simulink model "nmm2d"  (R2025a)
settings: Solver=ode15s  StartTime=0.0  StopTime=20  FixedStep=1e-3  MaxStep=ts_max  RelTol=1e-3  AbsTol=1e-4  EnableMultiTasking=on
values from neighbouring files (symbols this model uses):
  c = 0.05    [nmm2d_mInit.m]
  c_jointstop = 0.3 / (pi/180)    (= 17.1887338539)    [nmm2d_mInit.m]
  D12_F = 0.16    [nmm2d_mInit.m]
  D12_S = L_S    (= 0.5)    [nmm2d_mInit.m]
  D12_T = L_T    (= 0.5)    [nmm2d_mInit.m]
  D1G_F = 0.14    [nmm2d_mInit.m]
  D1G_HAT = 0.35    [nmm2d_mInit.m]
  D1G_S = 0.3    [nmm2d_mInit.m]
  D1G_T = 0.3    [nmm2d_mInit.m]
  DeltaThRef = 5e-3    (= 0.005)    [nmm2d_mInit.m]
  eref = 0.04    [nmm2d_mInit.m]
  FmaxVec = [FmaxSOL FmaxTA FmaxGAS FmaxVAS FmaxHAM FmaxGLU FmaxHFL               FmaxSOL FmaxTA FmaxGAS FmaxVAS FmaxHAM FmaxGLU FmaxHFL]'    [nmm2d_mInit.m]
  g = 9.81    [nmm2d_mInit.m]
  GainDeltaTheta = 2 /100*180/pi    (= 1.14591559026)    [nmm2d_cInit.m]
  GainGAS = 1.1/FmaxGAS    [nmm2d_cInit.m]
  GainGLU = 0.5/FmaxGLU    [nmm2d_cInit.m]
  GainHAM = 0.65/FmaxHAM    [nmm2d_cInit.m]
  GainHAMHFL = 4    [nmm2d_cInit.m]
  GainHFL = 0.5    [nmm2d_cInit.m]
  GainKneOverExt = 2    [nmm2d_cInit.m]
  GainSOL = 1.2/FmaxSOL    [nmm2d_cInit.m]
  GainSOLTA = 0.4/FmaxSOL    [nmm2d_cInit.m]
  GainTA = 1.1    [nmm2d_cInit.m]
  GainVAS = 1.2/FmaxVAS    [nmm2d_cInit.m]
  HAT_CG0 = [-D12_F; 0] + Rot120*[L_S;0] + Rot120*Rot230*[-L_T;0]            + Rot120*Rot230*Rot340*[D1G_HAT;0]    [nmm2d_cInit.m]
  In_F = 0.005    [nmm2d_mInit.m]
  In_HAT = 3    [nmm2d_mInit.m]
  In_S = 0.05    [nmm2d_mInit.m]
  In_T = 0.15    [nmm2d_mInit.m]
  K = 5    [nmm2d_mInit.m]
  k_gx = (2*(m_F+m_S+m_T)+m_HAT)*g/0.1    (= 7848)    [nmm2d_mInit.m]
  k_gy = (2*(m_F+m_S+m_T)+m_HAT)*g/0.01    (= 78480)    [nmm2d_mInit.m]
  k_pressure = m_HAT * 9.81 / DeltaThRef    (= 104967)    [nmm2d_mInit.m]
  K_swing = 0.25    [nmm2d_cInit.m]
  KneePh23Offset = 170*pi/180    (= 2.96705972839)    [nmm2d_cInit.m]
  L_F = 0.2    [nmm2d_mInit.m]
  L_HAT = 0.8    [nmm2d_mInit.m]
  L_S = 0.5    [nmm2d_mInit.m]
  L_T = 0.5    [nmm2d_mInit.m]
  LceOffsetHAM = 0.85    [nmm2d_cInit.m]
  LceOffsetHFL = 0.65    [nmm2d_cInit.m]
  LceOffsetTA = 1-0.5*w    [nmm2d_cInit.m]
  LongDelay = 0.020    (= 0.02)    [nmm2d_cInit.m]
  loptGAS = 0.05    [nmm2d_mInit.m]
  loptGLU = 0.11    [nmm2d_mInit.m]
  loptHAM = 0.10    (= 0.1)    [nmm2d_mInit.m]
  loptHFL = 0.11    [nmm2d_mInit.m]
  loptSOL = 0.04    [nmm2d_mInit.m]
  loptTA = 0.06    [nmm2d_mInit.m]
  loptVAS = 0.08    [nmm2d_mInit.m]
  loptVec = [loptSOL loptTA loptGAS loptVAS loptHAM loptGLU loptHFL               loptSOL loptTA loptGAS loptVAS loptHAM loptGLU loptHFL]'    [nmm2d_mInit.m]
  Lphi120 = 85*pi/180    (= 1.4835298642)    [nmm2d_cInit.m]
  Lphi230 = 175*pi/180    (= 3.05432619099)    [nmm2d_cInit.m]
  Lphi340 = 175*pi/180    (= 3.05432619099)    [nmm2d_cInit.m]
  lslackGAS = 0.40    (= 0.4)    [nmm2d_mInit.m]
  lslackGLU = 0.13    [nmm2d_mInit.m]
  lslackHAM = 0.31    [nmm2d_mInit.m]
  lslackHFL = 0.10    (= 0.1)    [nmm2d_mInit.m]
  lslackSOL = 0.26    [nmm2d_mInit.m]
  lslackTA = 0.24    [nmm2d_mInit.m]
  lslackVAS = 0.23    [nmm2d_mInit.m]
  lslackVec = [lslackSOL lslackTA lslackGAS lslackVAS lslackHAM lslackGLU lslackHFL                 lslackSOL lslackTA lslackGAS lslackVAS lslackHAM lslackGLU lslackHFL]'    [nmm2d_mInit.m]
  m_F = 1.25    [nmm2d_mInit.m]
  m_HAT = 53.5    [nmm2d_mInit.m]
  m_S = 3.5    [nmm2d_mInit.m]
  m_T = 8.5    [nmm2d_mInit.m]
  MidDelay = 0.010    (= 0.01)    [nmm2d_cInit.m]
  mu_slide = 0.8    [nmm2d_mInit.m]
  mu_stick = 0.9    [nmm2d_mInit.m]
  N = 1.5    [nmm2d_mInit.m]
  phi12_LowLimit = 70*pi/180    (= 1.2217304764)    [nmm2d_mInit.m]
  phi12_UpLimit = 130*pi/180    (= 2.26892802759)    [nmm2d_mInit.m]
  phi23_UpLimit = 175*pi/180    (= 3.05432619099)    [nmm2d_mInit.m]
  phi34_UpLimit = 230*pi/180    (= 4.01425727959)    [nmm2d_mInit.m]
  phimaxGASa = 110*pi/180    (= 1.91986217719)    [nmm2d_mInit.m]
  phimaxGASk = 140*pi/180    (= 2.44346095279)    [nmm2d_mInit.m]
  phimaxHAMk = 180*pi/180    (= 3.14159265359)    [nmm2d_mInit.m]
  phimaxSOL = 110*pi/180    (= 1.91986217719)    [nmm2d_mInit.m]
  phimaxTA = 80*pi/180    (= 1.3962634016)    [nmm2d_mInit.m]
  phimaxVAS = 165*pi/180    (= 2.87979326579)    [nmm2d_mInit.m]
  phirefGASa = 80*pi/180    (= 1.3962634016)    [nmm2d_mInit.m]
  phirefGASk = 165*pi/180    (= 2.87979326579)    [nmm2d_mInit.m]
  phirefGLU = 150*pi/180    (= 2.61799387799)    [nmm2d_mInit.m]
  phirefHAMh = 155*pi/180    (= 2.70526034059)    [nmm2d_mInit.m]
  phirefHAMk = 180*pi/180    (= 3.14159265359)    [nmm2d_mInit.m]
  phirefHFL = 180*pi/180    (= 3.14159265359)    [nmm2d_mInit.m]
  phirefSOL = 80*pi/180    (= 1.3962634016)    [nmm2d_mInit.m]
  phirefTA = 110*pi/180    (= 1.91986217719)    [nmm2d_mInit.m]
  phirefVAS = 125*pi/180    (= 2.18166156499)    [nmm2d_mInit.m]
  PosGainGG = 1/(30*pi/180)    (= 1.9098593171)    [nmm2d_cInit.m]
  preA = 0.01    [nmm2d_mInit.m]
  PreStimGAS = 0.01    [nmm2d_cInit.m]
  PreStimGG = 0.05    [nmm2d_cInit.m]
  PreStimGLU = 0.01    [nmm2d_cInit.m]
  PreStimHAM = 0.01    [nmm2d_cInit.m]
  PreStimHFL = 0.01    [nmm2d_cInit.m]
  PreStimSOL = 0.01    [nmm2d_cInit.m]
  PreStimTA = 0.01    [nmm2d_cInit.m]
  PreStimVAS = 0.08    [nmm2d_cInit.m]
  rGASa = 0.05    [nmm2d_mInit.m]
  rGASk = 0.05    [nmm2d_mInit.m]
  rGLU = 0.10    (= 0.1)    [nmm2d_mInit.m]
  rHAMh = 0.08    [nmm2d_mInit.m]
  rHAMk = 0.05    [nmm2d_mInit.m]
  rHFL = 0.10    (= 0.1)    [nmm2d_mInit.m]
  rhoGASa = 0.7    [nmm2d_mInit.m]
  rhoGASk = 0.7    [nmm2d_mInit.m]
  rhoGLU = 0.5    [nmm2d_mInit.m]
  rhoHAMh = 0.7    [nmm2d_mInit.m]
  rhoHAMk = 0.7    [nmm2d_mInit.m]
  rhoHFL = 0.5    [nmm2d_mInit.m]
  rhoSOL = 0.5    [nmm2d_mInit.m]
  rhoTA = 0.7    [nmm2d_mInit.m]
  rhoVAS = 0.7    [nmm2d_mInit.m]
  Rphi120 = 90*pi/180    (= 1.57079632679)    [nmm2d_cInit.m]
  Rphi230 = 175*pi/180    (= 3.05432619099)    [nmm2d_cInit.m]
  Rphi340 = 140*pi/180    (= 2.44346095279)    [nmm2d_cInit.m]
  rSOL = 0.05    [nmm2d_mInit.m]
  rTA = 0.04    [nmm2d_mInit.m]
  rVAS = 0.06    [nmm2d_mInit.m]
  ... (+12 more)
undefined symbols (not defined in the file or in its folder): sgn, X, Y, Z
libraries: sm_lib x70, nesl_utility x67, simulink x27, simulink_extras x6
(part 5 of 5)

== system nmm2d/Body Mechanics Layer/Right Ball Contact/Ground Friction Model ==
  note: Horizontal Ground Friction Model
  note: Vertical Ground Stiction Model
  dy [m] : Inport
  vy [m/s] : Inport  Port=2
  x [m] : Inport  Port=3
  vx [m/s] : Inport  Port=4
  vBelt [m/s] : Inport  Port=5
  Contact! : EnablePort  StatesWhenEnabling=reset
  Data Type Conversion : DataTypeConversion  OutDataTypeStr=double  SaturateOnIntegerOverflow=off  RndMeth=Floor
  Friction Switch : Subsystem
  Gain3 : Gain  Gain=k_gy
  Gain4 : Gain  Gain=1/v_gy_max
  Logical Operator : Logic  Operator=NOT  AllPortsSameDT=off  OutDataTypeStr=boolean
  Mux1 : Mux  Inputs=2
  Sum1 : Sum
  X-Axis Kinetic Friction Model : Subsystem
  X-Axis Static Friction Model : Subsystem
  Y-Axis Ground Force : Fcn  Expr="- u(1)  *  (1-u(2)) * (u(2)<1)"
  Fy_Ground[N] : Outport  OutputWhenDisabled=reset  InitialOutput=0
      settings: AttributesFormatString=initial = '%<InitialOutput>'\nwhen disabled = '%<OutputWhenDisabled>'
  Fx_Friction [N] : Outport  Port=2  OutputWhenDisabled=reset  InitialOutput=0
      settings: AttributesFormatString=initial = '%<InitialOutput>'\nwhen\ndisabled\n'%<OutputWhenDisabled>'
  Stiction! : Outport  Port=3  OutputWhenDisabled=reset  InitialOutput=0
      settings: AttributesFormatString=initial = '%<InitialOutput>'\nwhen\ndisabled\n'%<OutputWhenDisabled>'
  wires:
  Y-Axis Ground Force/1 -> X-Axis Kinetic Friction Model/4(F_Normal [N]), X-Axis Static Friction Model/1(F_Normal [N]), Fy_Ground[N]/1
  dy [m]/1 -> Gain3/1
  vy [m/s]/1 -> Gain4/1
  x [m]/1 -> X-Axis Kinetic Friction Model/1(pos [m]), X-Axis Static Friction Model/3(pos [m])
  vx [m/s]/1 -> X-Axis Static Friction Model/4(vel [m/s]), X-Axis Kinetic Friction Model/2(vel [m/s])
  X-Axis Kinetic Friction Model/1(initial posFP [m]) -> X-Axis Static Friction Model/5(initial posFP [m])
  X-Axis Kinetic Friction Model/3(F_Slide [N]) -> Sum1/2
  X-Axis Static Friction Model/1(F_Stick [N]) -> Sum1/1
  Sum1/1 -> Fx_Friction [N]/1
  Friction Switch/1(Stiction) -> X-Axis Static Friction Model/Enable, Logical Operator/1, Data Type Conversion/1
  X-Axis Static Friction Model/2(Sliding!) -> Friction Switch/1(Slide!)
  X-Axis Kinetic Friction Model/2(Stiction!) -> Friction Switch/2(Stick!)
  Logical Operator/1 -> X-Axis Kinetic Friction Model/Enable
  Data Type Conversion/1 -> Stiction!/1
  Mux1/1 -> Y-Axis Ground Force/1
  Gain3/1 -> Mux1/1
  Gain4/1 -> Mux1/2
  vBelt [m/s]/1 -> X-Axis Kinetic Friction Model/3(vBelt [m/s]), X-Axis Static Friction Model/2(vBelt [m/s])

== system nmm2d/Body Mechanics Layer/Right Heel Contact/Ground Friction Model ==
  note: Vertical Ground Stiction Model
  note: Horizontal Ground Friction Model
  dy [m] : Inport
  vy [m/s] : Inport  Port=2
  x [m] : Inport  Port=3
  vx [m/s] : Inport  Port=4
  vBelt [m/s] : Inport  Port=5
  Contact! : EnablePort  StatesWhenEnabling=reset
  Data Type Conversion : DataTypeConversion  OutDataTypeStr=double  SaturateOnIntegerOverflow=off  RndMeth=Floor
  Friction Switch : Subsystem
  Gain3 : Gain  Gain=k_gy
  Gain4 : Gain  Gain=1/v_gy_max
  Logical Operator : Logic  Operator=NOT  AllPortsSameDT=off  OutDataTypeStr=boolean
  Mux1 : Mux  Inputs=2
  Sum1 : Sum
  X-Axis Kinetic Friction Model : Subsystem
  X-Axis Static Friction Model : Subsystem
  Y-Axis Ground Force : Fcn  Expr="- u(1)  *  (1-u(2)) * (u(2)<1)"
  Fy_Ground[N] : Outport  OutputWhenDisabled=reset  InitialOutput=0
      settings: AttributesFormatString=initial = '%<InitialOutput>'\nwhen disabled = '%<OutputWhenDisabled>'
  Fx_Friction [N] : Outport  Port=2  OutputWhenDisabled=reset  InitialOutput=0
      settings: AttributesFormatString=initial = '%<InitialOutput>'\nwhen\ndisabled\n'%<OutputWhenDisabled>'
  Stiction! : Outport  Port=3  OutputWhenDisabled=reset  InitialOutput=0
      settings: AttributesFormatString=initial = '%<InitialOutput>'\nwhen\ndisabled\n'%<OutputWhenDisabled>'
  wires:
  vBelt [m/s]/1 -> X-Axis Static Friction Model/2(vBelt [m/s]), X-Axis Kinetic Friction Model/3(vBelt [m/s])
  Gain4/1 -> Mux1/2
  Gain3/1 -> Mux1/1
  Mux1/1 -> Y-Axis Ground Force/1
  Data Type Conversion/1 -> Stiction!/1
  Logical Operator/1 -> X-Axis Kinetic Friction Model/Enable
  X-Axis Kinetic Friction Model/2(Stiction!) -> Friction Switch/2(Stick!)
  X-Axis Static Friction Model/2(Sliding!) -> Friction Switch/1(Slide!)
  Friction Switch/1(Stiction) -> Data Type Conversion/1, Logical Operator/1, X-Axis Static Friction Model/Enable
  Sum1/1 -> Fx_Friction [N]/1
  X-Axis Static Friction Model/1(F_Stick [N]) -> Sum1/1
  X-Axis Kinetic Friction Model/3(F_Slide [N]) -> Sum1/2
  X-Axis Kinetic Friction Model/1(initial posFP [m]) -> X-Axis Static Friction Model/5(initial posFP [m])
  vx [m/s]/1 -> X-Axis Kinetic Friction Model/2(vel [m/s]), X-Axis Static Friction Model/4(vel [m/s])
  x [m]/1 -> X-Axis Static Friction Model/3(pos [m]), X-Axis Kinetic Friction Model/1(pos [m])
  vy [m/s]/1 -> Gain4/1
  dy [m]/1 -> Gain3/1
  Y-Axis Ground Force/1 -> Fy_Ground[N]/1, X-Axis Static Friction Model/1(F_Normal [N]), X-Axis Kinetic Friction Model/4(F_Normal [N])

== system nmm2d/Muscle Actuation Layer/VECTORIZED Muscle Dynamics/BE force-length relation ==
  note: Buffer Elasticity BE
  lce [lopt] : Inport
  Constant1 : Constant  Value=1-w
  Math Function : Math  Operator=square  SignedPower=on
  Sum4 : Sum  Inputs=|+-  InputSameDT=on  SaturateOnIntegerOverflow=on  OutDataTypeStr=Inherit: Same as first input
  buffer engaged? : simulink/Logic and Bit Operations/Compare To Zero  relop=<  OutDataTypeStr=boolean  ZeroCross=off
  force of buffer elasticity : Product  Inputs=**
  reference strain [lslack] : Constant  Value=w/2
  relative strain : Product  Inputs=*/
  fbe [Fmax] : Outport
  wires:
  force of buffer elasticity/1 -> fbe [Fmax]/1
  Math Function/1 -> force of buffer elasticity/2
  buffer engaged?/1 -> force of buffer elasticity/1
  Constant1/1 -> Sum4/2
  Sum4/1 -> relative strain/1, buffer engaged?/1
  reference strain [lslack]/1 -> relative strain/2
  relative strain/1 -> Math Function/1
  lce [lopt]/1 -> Sum4/1

== system nmm2d/Muscle Actuation Layer/VECTORIZED Muscle Dynamics/CE force-length relation ==
  note: CE Force-Length Relationship
  lce [lopt] : Inport
  Abs : Abs  SaturateOnIntegerOverflow=off
  Constant1 : Constant
  Constant2 : Constant  Value=3
  Gain : Gain  Gain=log(c)
  Math Function : Math  SignedPower=on
  Math Function1 : Math  Operator=pow  SignedPower=on
  Sum4 : Sum  Inputs=|+-  InputSameDT=on  SaturateOnIntegerOverflow=on  OutDataTypeStr=Inherit: Same as first input
  normalized position : Product  Inputs=*/
  relative width : Constant  Value=w
  fce [Fmax] : Outport
  wires:
  Math Function/1 -> fce [Fmax]/1
  Gain/1 -> Math Function/1
  Math Function1/1 -> Gain/1
  Constant2/1 -> Math Function1/2
  normalized position/1 -> Math Function1/1
  Abs/1 -> normalized position/1
  Sum4/1 -> Abs/1
  Constant1/1 -> Sum4/2
  relative width/1 -> normalized position/2
  lce [lopt]/1 -> Sum4/1

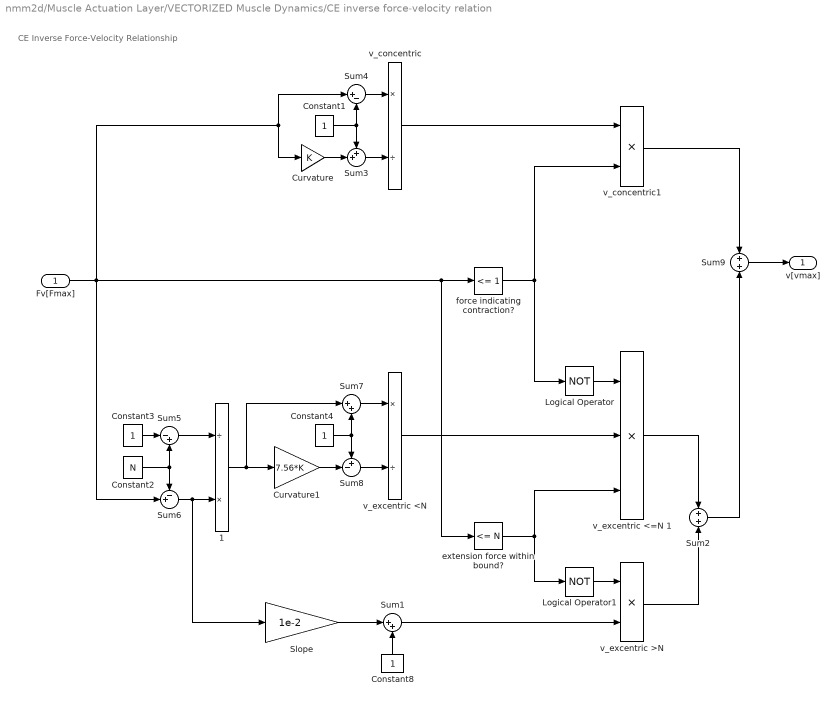
== system nmm2d/Muscle Actuation Layer/VECTORIZED Muscle Dynamics/CE inverse force-velocity relation ==
  note: CE Inverse Force-Velocity Relationship
  Fv[Fmax] : Inport
  1 : Product  Inputs=/*
  Constant{1,3..4,8} (4 alike) : Constant
  Constant2 : Constant  Value=N
  Curvature : Gain  Gain=K  SaturateOnIntegerOverflow=on  OutDataTypeStr=Inherit: Same as input  ParamDataTypeStr=Inherit: Same as input
  Curvature1 : Gain  Gain=7.56*K  SaturateOnIntegerOverflow=on  OutDataTypeStr=Inherit: Same as input  ParamDataTypeStr=Inherit: Same as input
  Logical Operator : Logic  Operator=NOT  AllPortsSameDT=off  OutDataTypeStr=boolean
  Logical Operator1 : Logic  Operator=NOT  AllPortsSameDT=off  OutDataTypeStr=boolean
  Slope : Gain  Gain=1e-2  SaturateOnIntegerOverflow=on  OutDataTypeStr=Inherit: Same as input  ParamDataTypeStr=Inherit: Same as input
  Sum1 : Sum  Inputs=|++  InputSameDT=on  SaturateOnIntegerOverflow=on  OutDataTypeStr=Inherit: Same as first input
  Sum2 : Sum  InputSameDT=on  SaturateOnIntegerOverflow=on  OutDataTypeStr=Inherit: Same as first input
  Sum3 : Sum  Inputs=++|  InputSameDT=on  SaturateOnIntegerOverflow=on  OutDataTypeStr=Inherit: Same as first input
  Sum4 : Sum  Inputs=|+-  InputSameDT=on  SaturateOnIntegerOverflow=on  OutDataTypeStr=Inherit: Same as first input
  Sum5 : Sum  Inputs=|-+  InputSameDT=on  SaturateOnIntegerOverflow=on  OutDataTypeStr=Inherit: Same as first input
  Sum6 : Sum  Inputs=-+|  InputSameDT=on  SaturateOnIntegerOverflow=on  OutDataTypeStr=Inherit: Same as first input
  Sum7 : Sum  Inputs=|++  InputSameDT=on  SaturateOnIntegerOverflow=on  OutDataTypeStr=Inherit: Same as first input
  Sum8 : Sum  Inputs=+-|  InputSameDT=on  SaturateOnIntegerOverflow=on  OutDataTypeStr=Inherit: Same as first input
  Sum9 : Sum  InputSameDT=on  SaturateOnIntegerOverflow=on  OutDataTypeStr=Inherit: Same as first input
  extension force within bound? : simulink/Logic and Bit Operations/Compare To Constant  relop=<=  const=N  OutDataTypeStr=boolean  ZeroCross=off
  force indicating contraction? : simulink/Logic and Bit Operations/Compare To Constant  relop=<=  const=1  OutDataTypeStr=boolean  ZeroCross=off
  v_concentric : Product  Inputs=*/
  v_concentric1 : Product  Inputs=**
  v_excentric <=N 1 : Product  Inputs=***
  v_excentric <N : Product  Inputs=*/
  v_excentric >N : Product  Inputs=**
  v[vmax] : Outport
  wires:
  Sum2/1 -> Sum9/2
  v_excentric <=N 1/1 -> Sum2/1
  Logical Operator1/1 -> v_excentric >N/1
  v_excentric >N/1 -> Sum2/2
  Logical Operator/1 -> v_excentric <=N 1/1
  Fv[Fmax]/1 -> Sum6/2, extension force within bound?/1, force indicating contraction?/1, Curvature/1, Sum4/1
  extension force within bound?/1 -> Logical Operator1/1, v_excentric <=N 1/3
  force indicating contraction?/1 -> Logical Operator/1, v_concentric1/2
  Sum1/1 -> v_excentric >N/2
  v_concentric1/1 -> Sum9/1
  v_excentric <N/1 -> v_excentric <=N 1/2
  Constant3/1 -> Sum5/1
  Sum5/1 -> 1/1
  Constant2/1 -> Sum5/2, Sum6/1
  Sum6/1 -> Slope/1, 1/2
  Constant8/1 -> Sum1/2
  Slope/1 -> Sum1/1
  Sum9/1 -> v[vmax]/1
  v_concentric/1 -> v_concentric1/1
  Sum7/1 -> v_excentric <N/1
  Sum8/1 -> v_excentric <N/2
  Curvature1/1 -> Sum8/2
  Constant4/1 -> Sum8/1, Sum7/2
  1/1 -> Curvature1/1, Sum7/1
  Sum3/1 -> v_concentric/2
  Sum4/1 -> v_concentric/1
  Constant1/1 -> Sum3/1, Sum4/2
  Curvature/1 -> Sum3/2

== system nmm2d/Muscle Actuation Layer/VECTORIZED Muscle Dynamics/PE force-length relation ==
  note: Parallel Elasticity PE
  lce [lopt] : Inport
  Constant3 : Constant
  Math Function2 : Math  Operator=square  SignedPower=on
  Sum1 : Sum  Inputs=|+-  InputSameDT=on  SaturateOnIntegerOverflow=on  OutDataTypeStr=Inherit: Same as first input
  force of buffer elasticity : Product  Inputs=**
  parallel elasticity engaged? : simulink/Logic and Bit Operations/Compare To Zero  relop=>  OutDataTypeStr=boolean  ZeroCross=off
  reference strain [lopt] : Constant  Value=w
  relative strain : Product  Inputs=*/
  fpe [Fmax] : Outport
  wires:
  parallel elasticity engaged?/1 -> force of buffer elasticity/1
  force of buffer elasticity/1 -> fpe [Fmax]/1
  Math Function2/1 -> force of buffer elasticity/2
  relative strain/1 -> Math Function2/1
  reference strain [lopt]/1 -> relative strain/2
  Sum1/1 -> relative strain/1, parallel elasticity engaged?/1
  Constant3/1 -> Sum1/2
  lce [lopt]/1 -> Sum1/1

== system nmm2d/Muscle Actuation Layer/VECTORIZED Muscle Dynamics/SE force-length relation ==
  note: SE Force-Length Relationship
  lse [lslack] : Inport
  Constant1 : Constant
  Math Function : Math  Operator=square  SignedPower=on
  Sum4 : Sum  Inputs=|+-  InputSameDT=on  SaturateOnIntegerOverflow=on  OutDataTypeStr=Inherit: Same as first input
  force above slack length : Product  Inputs=**
  greater than slack length? : simulink/Logic and Bit Operations/Compare To Zero  relop=>  OutDataTypeStr=boolean  ZeroCross=off
  reference strain [lslack] : Constant  Value=eref
  relative strain : Product  Inputs=*/
  fse [Fmax] : Outport
  wires:
  force above slack length/1 -> fse [Fmax]/1
  greater than slack length?/1 -> force above slack length/1
  Constant1/1 -> Sum4/2
  Sum4/1 -> relative strain/1, greater than slack length?/1
  reference strain [lslack]/1 -> relative strain/2
  relative strain/1 -> Math Function/1
  lse [lslack]/1 -> Sum4/1
  Math Function/1 -> force above slack length/2

== system nmm2d/Body Mechanics Layer/Left Ball Contact/Ground Friction Model/Friction Switch ==
  note: Static/Kinetic Friction Switch
  Slide! : Inport
  Stick! : Inport  Port=2
  Memory : Memory
  S-R Flip-Flop : simulink_extras/Flip Flops/S-R Flip-Flop  initial_condition=1
  Terminator : Terminator
  Stiction : Outport
  wires:
  S-R Flip-Flop/1 -> Memory/1
  S-R Flip-Flop/2 -> Terminator/1
  Stick!/1 -> S-R Flip-Flop/1
  Slide!/1 -> S-R Flip-Flop/2
  Memory/1 -> Stiction/1

== system nmm2d/Body Mechanics Layer/Left Ball Contact/Ground Friction Model/X-Axis Kinetic Friction Model ==
  note: Kinetic Friction Model
  note: Footpoint Determiner
  note: Sliding Limit Detector
  pos [m] : Inport
  vel [m/s] : Inport  Port=2
  vBelt [m/s] : Inport  Port=3
  F_Normal [N] : Inport  Port=4
  Enable : EnablePort  StatesWhenEnabling=reset  ZeroCross=off
  Abs : Abs  SaturateOnIntegerOverflow=off
  Constant : Constant  Value=vLimit
  FixPt Relational Operator : RelationalOperator  Operator=>  OutDataTypeStr=boolean  ZeroCross=off  InputSameDT=off
  Memory : Memory
  Negative : simulink/Logic and Bit Operations/Compare To Zero  relop=<  OutDataTypeStr=boolean
  Product : Product  RndMeth=Zero
  Sign1 : Signum
  Sum : Sum  Inputs=|+-
  Sum1 : Sum  Inputs=|+-
  reverse : Gain  Gain=-1
  sliding friction coefficient : Gain  Gain=mu_slide
  initial posFP [m] : Outport  InitialOutput=0
      settings: AttributesFormatString=initial = '%<InitialOutput>'\nwhen disabled = '%<OutputWhenDisabled>'
  Stiction! : Outport  Port=2  OutputWhenDisabled=reset  InitialOutput=0
      settings: AttributesFormatString=initial = '%<InitialOutput>'\nwhen disabled = '%<OutputWhenDisabled>'
  F_Slide [N] : Outport  Port=3  OutputWhenDisabled=reset  InitialOutput=0
      settings: AttributesFormatString=initial = '%<InitialOutput>'\nwhen disabled = '%<OutputWhenDisabled>'
  wires:
  reverse/1 -> Product/1
  F_Normal [N]/1 -> sliding friction coefficient/1
  Sum1/1 -> Sign1/1, Abs/1
  pos [m]/1 -> initial posFP [m]/1
  Product/1 -> F_Slide [N]/1
  sliding friction coefficient/1 -> Product/2
  Sign1/1 -> reverse/1
  FixPt Relational Operator/1 -> Stiction!/1
  Memory/1 -> FixPt Relational Operator/2
  Negative/1 -> FixPt Relational Operator/1, Memory/1
  Abs/1 -> Sum/1
  Sum/1 -> Negative/1
  Constant/1 -> Sum/2
  vel [m/s]/1 -> Sum1/1
  vBelt [m/s]/1 -> Sum1/2

== system nmm2d/Body Mechanics Layer/Left Ball Contact/Ground Friction Model/X-Axis Static Friction Model ==
  note: Zero multiplication prevents
      | horizontal friction model from
      | oscillating between static and kinetic
      | friction when the vertical force is zero but
      | the ground level is not yet reached
      | in the upward motion
  note: Stiction Limit Detector
  note: Static Friction Model
  F_Normal [N] : Inport
  vBelt [m/s] : Inport  Port=2
  pos [m] : Inport  Port=3
  vel [m/s] : Inport  Port=4
  initial posFP [m] : Inport  Port=5
  Enable : EnablePort  StatesWhenEnabling=reset  ZeroCross=off
  Abs : Abs  SaturateOnIntegerOverflow=off
  Abs. : Abs  SaturateOnIntegerOverflow=off
  Check Vertical Friction : Product  RndMeth=Zero
  FixPt Relational Operator : RelationalOperator  Operator=>  OutDataTypeStr=boolean  ZeroCross=off  InputSameDT=off
  Gain3 : Gain  Gain=k_gx
  Gain4 : Gain  Gain=1/v_gx_max
  Integrator : Integrator  InitialConditionSource=external
  Memory : Memory
  Mux1 : Mux  Inputs=2
  Positive : simulink/Logic and Bit Operations/Compare To Zero  relop=>  OutDataTypeStr=boolean
  Positive1 : simulink/Logic and Bit Operations/Compare To Zero  relop=>  OutDataTypeStr=boolean
  Sum : Sum  Inputs=-+
  Sum1 : Sum  Inputs=-+|
  Sum2 : Sum  Inputs=-+|
  X-Axis Stiction Force : Fcn  Expr=-u(1) * (1+sgn(u(1))*u(2))
  stiction limit force : Gain  Gain=mu_stick
  F_Stick [N] : Outport  OutputWhenDisabled=reset  InitialOutput=0
      settings: AttributesFormatString=when disabled: %<OutputWhenDisabled>\ninitial: %<InitialOutput>
  Sliding! : Outport  Port=2  OutputWhenDisabled=reset  InitialOutput=0
      settings: AttributesFormatString=when disabled: %<OutputWhenDisabled>\ninitial: %<InitialOutput>
  wires:
  Check Vertical Friction/1 -> Abs./1, F_Stick [N]/1
  Positive1/1 -> Check Vertical Friction/2
  X-Axis Stiction Force/1 -> Check Vertical Friction/1
  stiction limit force/1 -> Abs/1
  Abs/1 -> Sum/1
  FixPt Relational Operator/1 -> Sliding!/1
  Gain4/1 -> Mux1/2
  Gain3/1 -> Mux1/1
  Mux1/1 -> X-Axis Stiction Force/1
  Abs./1 -> Sum/2
  Positive/1 -> Memory/1, FixPt Relational Operator/1
  Memory/1 -> FixPt Relational Operator/2
  Sum/1 -> Positive/1
  pos [m]/1 -> Sum2/2
  Sum2/1 -> Gain3/1  "dx"
  F_Normal [N]/1 -> Positive1/1, stiction limit force/1
  initial posFP [m]/1 -> Integrator/2
  vBelt [m/s]/1 -> Sum1/1, Integrator/1
  Integrator/1 -> Sum2/1  "xFP"
  vel [m/s]/1 -> Sum1/2
  Sum1/1 -> Gain4/1  "dx"

== system nmm2d/Body Mechanics Layer/Left Heel Contact/Ground Friction Model/Friction Switch ==
  note: Static/Kinetic Friction Switch
  Slide! : Inport
  Stick! : Inport  Port=2
  Memory : Memory
  S-R Flip-Flop : simulink_extras/Flip Flops/S-R Flip-Flop  initial_condition=1
  Terminator : Terminator
  Stiction : Outport
  wires:
  Memory/1 -> Stiction/1
  Slide!/1 -> S-R Flip-Flop/2
  Stick!/1 -> S-R Flip-Flop/1
  S-R Flip-Flop/2 -> Terminator/1
  S-R Flip-Flop/1 -> Memory/1

== system nmm2d/Body Mechanics Layer/Left Heel Contact/Ground Friction Model/X-Axis Kinetic Friction Model ==
  note: Sliding Limit Detector
  note: Footpoint Determiner
  note: Kinetic Friction Model
  pos [m] : Inport
  vel [m/s] : Inport  Port=2
  vBelt [m/s] : Inport  Port=3
  F_Normal [N] : Inport  Port=4
  Enable : EnablePort  StatesWhenEnabling=reset  ZeroCross=off
  Abs : Abs  SaturateOnIntegerOverflow=off
  Constant : Constant  Value=vLimit
  FixPt Relational Operator : RelationalOperator  Operator=>  OutDataTypeStr=boolean  ZeroCross=off  InputSameDT=off
  Memory : Memory
  Negative : simulink/Logic and Bit Operations/Compare To Zero  relop=<  OutDataTypeStr=boolean
  Product : Product  RndMeth=Zero
  Sign1 : Signum
  Sum : Sum  Inputs=|+-
  Sum1 : Sum  Inputs=|+-
  reverse : Gain  Gain=-1
  sliding friction coefficient : Gain  Gain=mu_slide
  initial posFP [m] : Outport  InitialOutput=0
      settings: AttributesFormatString=initial = '%<InitialOutput>'\nwhen disabled = '%<OutputWhenDisabled>'
  Stiction! : Outport  Port=2  OutputWhenDisabled=reset  InitialOutput=0
      settings: AttributesFormatString=initial = '%<InitialOutput>'\nwhen disabled = '%<OutputWhenDisabled>'
  F_Slide [N] : Outport  Port=3  OutputWhenDisabled=reset  InitialOutput=0
      settings: AttributesFormatString=initial = '%<InitialOutput>'\nwhen disabled = '%<OutputWhenDisabled>'
  wires:
  vBelt [m/s]/1 -> Sum1/2
  vel [m/s]/1 -> Sum1/1
  Constant/1 -> Sum/2
  Sum/1 -> Negative/1
  Abs/1 -> Sum/1
  Negative/1 -> Memory/1, FixPt Relational Operator/1
  Memory/1 -> FixPt Relational Operator/2
  FixPt Relational Operator/1 -> Stiction!/1
  Sign1/1 -> reverse/1
  sliding friction coefficient/1 -> Product/2
  Product/1 -> F_Slide [N]/1
  pos [m]/1 -> initial posFP [m]/1
  Sum1/1 -> Abs/1, Sign1/1
  F_Normal [N]/1 -> sliding friction coefficient/1
  reverse/1 -> Product/1

== system nmm2d/Body Mechanics Layer/Left Heel Contact/Ground Friction Model/X-Axis Static Friction Model ==
  note: Static Friction Model
  note: Stiction Limit Detector
  note: Zero multiplication prevents
      | horizontal friction model from
      | oscillating between static and kinetic
      | friction when the vertical force is zero but
      | the ground level is not yet reached
      | in the upward motion
  F_Normal [N] : Inport
  vBelt [m/s] : Inport  Port=2
  pos [m] : Inport  Port=3
  vel [m/s] : Inport  Port=4
  initial posFP [m] : Inport  Port=5
  Enable : EnablePort  StatesWhenEnabling=reset  ZeroCross=off
  Abs : Abs  SaturateOnIntegerOverflow=off
  Abs. : Abs  SaturateOnIntegerOverflow=off
  Check Vertical Friction : Product  RndMeth=Zero
  FixPt Relational Operator : RelationalOperator  Operator=>  OutDataTypeStr=boolean  ZeroCross=off  InputSameDT=off
  Gain3 : Gain  Gain=k_gx
  Gain4 : Gain  Gain=1/v_gx_max
  Integrator : Integrator  InitialConditionSource=external
  Memory : Memory
  Mux1 : Mux  Inputs=2
  Positive : simulink/Logic and Bit Operations/Compare To Zero  relop=>  OutDataTypeStr=boolean
  Positive1 : simulink/Logic and Bit Operations/Compare To Zero  relop=>  OutDataTypeStr=boolean
  Sum : Sum  Inputs=-+
  Sum1 : Sum  Inputs=-+|
  Sum2 : Sum  Inputs=-+|
  X-Axis Stiction Force : Fcn  Expr=-u(1) * (1+sgn(u(1))*u(2))
  stiction limit force : Gain  Gain=mu_stick
  F_Stick [N] : Outport  OutputWhenDisabled=reset  InitialOutput=0
      settings: AttributesFormatString=when disabled: %<OutputWhenDisabled>\ninitial: %<InitialOutput>
  Sliding! : Outport  Port=2  OutputWhenDisabled=reset  InitialOutput=0
      settings: AttributesFormatString=when disabled: %<OutputWhenDisabled>\ninitial: %<InitialOutput>
  wires:
  Sum1/1 -> Gain4/1  "dx"
  vel [m/s]/1 -> Sum1/2
  Integrator/1 -> Sum2/1  "xFP"
  vBelt [m/s]/1 -> Integrator/1, Sum1/1
  initial posFP [m]/1 -> Integrator/2
  F_Normal [N]/1 -> stiction limit force/1, Positive1/1
  Sum2/1 -> Gain3/1  "dx"
  pos [m]/1 -> Sum2/2
  Sum/1 -> Positive/1
  Memory/1 -> FixPt Relational Operator/2
  Positive/1 -> FixPt Relational Operator/1, Memory/1
  Abs./1 -> Sum/2
  Mux1/1 -> X-Axis Stiction Force/1
  Gain3/1 -> Mux1/1
  Gain4/1 -> Mux1/2
  FixPt Relational Operator/1 -> Sliding!/1
  Abs/1 -> Sum/1
  stiction limit force/1 -> Abs/1
  X-Axis Stiction Force/1 -> Check Vertical Friction/1
  Positive1/1 -> Check Vertical Friction/2
  Check Vertical Friction/1 -> F_Stick [N]/1, Abs./1

== system nmm2d/Body Mechanics Layer/Right Ball Contact/Ground Friction Model/Friction Switch ==
  note: Static/Kinetic Friction Switch
  Slide! : Inport
  Stick! : Inport  Port=2
  Memory : Memory
  S-R Flip-Flop : simulink_extras/Flip Flops/S-R Flip-Flop  initial_condition=1
  Terminator : Terminator
  Stiction : Outport
  wires:
  S-R Flip-Flop/1 -> Memory/1
  S-R Flip-Flop/2 -> Terminator/1
  Stick!/1 -> S-R Flip-Flop/1
  Slide!/1 -> S-R Flip-Flop/2
  Memory/1 -> Stiction/1

== system nmm2d/Body Mechanics Layer/Right Ball Contact/Ground Friction Model/X-Axis Kinetic Friction Model ==
  note: Kinetic Friction Model
  note: Footpoint Determiner
  note: Sliding Limit Detector
  pos [m] : Inport
  vel [m/s] : Inport  Port=2
  vBelt [m/s] : Inport  Port=3
  F_Normal [N] : Inport  Port=4
  Enable : EnablePort  StatesWhenEnabling=reset  ZeroCross=off
  Abs : Abs  SaturateOnIntegerOverflow=off
  Constant : Constant  Value=vLimit
  FixPt Relational Operator : RelationalOperator  Operator=>  OutDataTypeStr=boolean  ZeroCross=off  InputSameDT=off
  Memory : Memory
  Negative : simulink/Logic and Bit Operations/Compare To Zero  relop=<  OutDataTypeStr=boolean
  Product : Product  RndMeth=Zero
  Sign1 : Signum
  Sum : Sum  Inputs=|+-
  Sum1 : Sum  Inputs=|+-
  reverse : Gain  Gain=-1
  sliding friction coefficient : Gain  Gain=mu_slide
  initial posFP [m] : Outport  InitialOutput=0
      settings: AttributesFormatString=initial = '%<InitialOutput>'\nwhen disabled = '%<OutputWhenDisabled>'
  Stiction! : Outport  Port=2  OutputWhenDisabled=reset  InitialOutput=0
      settings: AttributesFormatString=initial = '%<InitialOutput>'\nwhen disabled = '%<OutputWhenDisabled>'
  F_Slide [N] : Outport  Port=3  OutputWhenDisabled=reset  InitialOutput=0
      settings: AttributesFormatString=initial = '%<InitialOutput>'\nwhen disabled = '%<OutputWhenDisabled>'
  wires:
  reverse/1 -> Product/1
  F_Normal [N]/1 -> sliding friction coefficient/1
  Sum1/1 -> Sign1/1, Abs/1
  pos [m]/1 -> initial posFP [m]/1
  Product/1 -> F_Slide [N]/1
  sliding friction coefficient/1 -> Product/2
  Sign1/1 -> reverse/1
  FixPt Relational Operator/1 -> Stiction!/1
  Memory/1 -> FixPt Relational Operator/2
  Negative/1 -> FixPt Relational Operator/1, Memory/1
  Abs/1 -> Sum/1
  Sum/1 -> Negative/1
  Constant/1 -> Sum/2
  vel [m/s]/1 -> Sum1/1
  vBelt [m/s]/1 -> Sum1/2

== system nmm2d/Body Mechanics Layer/Right Ball Contact/Ground Friction Model/X-Axis Static Friction Model ==
  note: Zero multiplication prevents
      | horizontal friction model from
      | oscillating between static and kinetic
      | friction when the vertical force is zero but
      | the ground level is not yet reached
      | in the upward motion
  note: Stiction Limit Detector
  note: Static Friction Model
  F_Normal [N] : Inport
  vBelt [m/s] : Inport  Port=2
  pos [m] : Inport  Port=3
  vel [m/s] : Inport  Port=4
  initial posFP [m] : Inport  Port=5
  Enable : EnablePort  StatesWhenEnabling=reset  ZeroCross=off
  Abs : Abs  SaturateOnIntegerOverflow=off
  Abs. : Abs  SaturateOnIntegerOverflow=off
  Check Vertical Friction : Product  RndMeth=Zero
  FixPt Relational Operator : RelationalOperator  Operator=>  OutDataTypeStr=boolean  ZeroCross=off  InputSameDT=off
  Gain3 : Gain  Gain=k_gx
  Gain4 : Gain  Gain=1/v_gx_max
  Integrator : Integrator  InitialConditionSource=external
  Memory : Memory
  Mux1 : Mux  Inputs=2
  Positive : simulink/Logic and Bit Operations/Compare To Zero  relop=>  OutDataTypeStr=boolean
  Positive1 : simulink/Logic and Bit Operations/Compare To Zero  relop=>  OutDataTypeStr=boolean
  Sum : Sum  Inputs=-+
  Sum1 : Sum  Inputs=-+|
  Sum2 : Sum  Inputs=-+|
  X-Axis Stiction Force : Fcn  Expr=-u(1) * (1+sgn(u(1))*u(2))
  stiction limit force : Gain  Gain=mu_stick
  F_Stick [N] : Outport  OutputWhenDisabled=reset  InitialOutput=0
      settings: AttributesFormatString=when disabled: %<OutputWhenDisabled>\ninitial: %<InitialOutput>
  Sliding! : Outport  Port=2  OutputWhenDisabled=reset  InitialOutput=0
      settings: AttributesFormatString=when disabled: %<OutputWhenDisabled>\ninitial: %<InitialOutput>
  wires:
  Check Vertical Friction/1 -> Abs./1, F_Stick [N]/1
  Positive1/1 -> Check Vertical Friction/2
  X-Axis Stiction Force/1 -> Check Vertical Friction/1
  stiction limit force/1 -> Abs/1
  Abs/1 -> Sum/1
  FixPt Relational Operator/1 -> Sliding!/1
  Gain4/1 -> Mux1/2
  Gain3/1 -> Mux1/1
  Mux1/1 -> X-Axis Stiction Force/1
  Abs./1 -> Sum/2
  Positive/1 -> Memory/1, FixPt Relational Operator/1
  Memory/1 -> FixPt Relational Operator/2
  Sum/1 -> Positive/1
  pos [m]/1 -> Sum2/2
  Sum2/1 -> Gain3/1  "dx"
  F_Normal [N]/1 -> Positive1/1, stiction limit force/1
  initial posFP [m]/1 -> Integrator/2
  vBelt [m/s]/1 -> Sum1/1, Integrator/1
  Integrator/1 -> Sum2/1  "xFP"
  vel [m/s]/1 -> Sum1/2
  Sum1/1 -> Gain4/1  "dx"

== system nmm2d/Body Mechanics Layer/Right Heel Contact/Ground Friction Model/Friction Switch ==
  note: Static/Kinetic Friction Switch
  Slide! : Inport
  Stick! : Inport  Port=2
  Memory : Memory
  S-R Flip-Flop : simulink_extras/Flip Flops/S-R Flip-Flop  initial_condition=1
  Terminator : Terminator
  Stiction : Outport
  wires:
  Memory/1 -> Stiction/1
  Slide!/1 -> S-R Flip-Flop/2
  Stick!/1 -> S-R Flip-Flop/1
  S-R Flip-Flop/2 -> Terminator/1
  S-R Flip-Flop/1 -> Memory/1

== system nmm2d/Body Mechanics Layer/Right Heel Contact/Ground Friction Model/X-Axis Kinetic Friction Model ==
  note: Sliding Limit Detector
  note: Footpoint Determiner
  note: Kinetic Friction Model
  pos [m] : Inport
  vel [m/s] : Inport  Port=2
  vBelt [m/s] : Inport  Port=3
  F_Normal [N] : Inport  Port=4
  Enable : EnablePort  StatesWhenEnabling=reset  ZeroCross=off
  Abs : Abs  SaturateOnIntegerOverflow=off
  Constant : Constant  Value=vLimit
  FixPt Relational Operator : RelationalOperator  Operator=>  OutDataTypeStr=boolean  ZeroCross=off  InputSameDT=off
  Memory : Memory
  Negative : simulink/Logic and Bit Operations/Compare To Zero  relop=<  OutDataTypeStr=boolean
  Product : Product  RndMeth=Zero
  Sign1 : Signum
  Sum : Sum  Inputs=|+-
  Sum1 : Sum  Inputs=|+-
  reverse : Gain  Gain=-1
  sliding friction coefficient : Gain  Gain=mu_slide
  initial posFP [m] : Outport  InitialOutput=0
      settings: AttributesFormatString=initial = '%<InitialOutput>'\nwhen disabled = '%<OutputWhenDisabled>'
  Stiction! : Outport  Port=2  OutputWhenDisabled=reset  InitialOutput=0
      settings: AttributesFormatString=initial = '%<InitialOutput>'\nwhen disabled = '%<OutputWhenDisabled>'
  F_Slide [N] : Outport  Port=3  OutputWhenDisabled=reset  InitialOutput=0
      settings: AttributesFormatString=initial = '%<InitialOutput>'\nwhen disabled = '%<OutputWhenDisabled>'
  wires:
  vBelt [m/s]/1 -> Sum1/2
  vel [m/s]/1 -> Sum1/1
  Constant/1 -> Sum/2
  Sum/1 -> Negative/1
  Abs/1 -> Sum/1
  Negative/1 -> Memory/1, FixPt Relational Operator/1
  Memory/1 -> FixPt Relational Operator/2
  FixPt Relational Operator/1 -> Stiction!/1
  Sign1/1 -> reverse/1
  sliding friction coefficient/1 -> Product/2
  Product/1 -> F_Slide [N]/1
  pos [m]/1 -> initial posFP [m]/1
  Sum1/1 -> Abs/1, Sign1/1
  F_Normal [N]/1 -> sliding friction coefficient/1
  reverse/1 -> Product/1

== system nmm2d/Body Mechanics Layer/Right Heel Contact/Ground Friction Model/X-Axis Static Friction Model ==
  note: Static Friction Model
  note: Stiction Limit Detector
  note: Zero multiplication prevents
      | horizontal friction model from
      | oscillating between static and kinetic
      | friction when the vertical force is zero but
      | the ground level is not yet reached
      | in the upward motion
  F_Normal [N] : Inport
  vBelt [m/s] : Inport  Port=2
  pos [m] : Inport  Port=3
  vel [m/s] : Inport  Port=4
  initial posFP [m] : Inport  Port=5
  Enable : EnablePort  StatesWhenEnabling=reset  ZeroCross=off
  Abs : Abs  SaturateOnIntegerOverflow=off
  Abs. : Abs  SaturateOnIntegerOverflow=off
  Check Vertical Friction : Product  RndMeth=Zero
  FixPt Relational Operator : RelationalOperator  Operator=>  OutDataTypeStr=boolean  ZeroCross=off  InputSameDT=off
  Gain3 : Gain  Gain=k_gx
  Gain4 : Gain  Gain=1/v_gx_max
  Integrator : Integrator  InitialConditionSource=external
  Memory : Memory
  Mux1 : Mux  Inputs=2
  Positive : simulink/Logic and Bit Operations/Compare To Zero  relop=>  OutDataTypeStr=boolean
  Positive1 : simulink/Logic and Bit Operations/Compare To Zero  relop=>  OutDataTypeStr=boolean
  Sum : Sum  Inputs=-+
  Sum1 : Sum  Inputs=-+|
  Sum2 : Sum  Inputs=-+|
  X-Axis Stiction Force : Fcn  Expr=-u(1) * (1+sgn(u(1))*u(2))
  stiction limit force : Gain  Gain=mu_stick
  F_Stick [N] : Outport  OutputWhenDisabled=reset  InitialOutput=0
      settings: AttributesFormatString=when disabled: %<OutputWhenDisabled>\ninitial: %<InitialOutput>
  Sliding! : Outport  Port=2  OutputWhenDisabled=reset  InitialOutput=0
      settings: AttributesFormatString=when disabled: %<OutputWhenDisabled>\ninitial: %<InitialOutput>
  wires:
  Sum1/1 -> Gain4/1  "dx"
  vel [m/s]/1 -> Sum1/2
  Integrator/1 -> Sum2/1  "xFP"
  vBelt [m/s]/1 -> Integrator/1, Sum1/1
  initial posFP [m]/1 -> Integrator/2
  F_Normal [N]/1 -> stiction limit force/1, Positive1/1
  Sum2/1 -> Gain3/1  "dx"
  pos [m]/1 -> Sum2/2
  Sum/1 -> Positive/1
  Memory/1 -> FixPt Relational Operator/2
  Positive/1 -> FixPt Relational Operator/1, Memory/1
  Abs./1 -> Sum/2
  Mux1/1 -> X-Axis Stiction Force/1
  Gain3/1 -> Mux1/1
  Gain4/1 -> Mux1/2
  FixPt Relational Operator/1 -> Sliding!/1
  Abs/1 -> Sum/1
  stiction limit force/1 -> Abs/1
  X-Axis Stiction Force/1 -> Check Vertical Friction/1
  Positive1/1 -> Check Vertical Friction/2
  Check Vertical Friction/1 -> F_Stick [N]/1, Abs./1
